simulink model "single_phase_multilevel_sm"  (R2026a)
settings: Solver=ode1be  StopTime=simlength  FixedStep=tc
values from neighbouring files (symbols this model uses):
  Vfc1_base = Udc/5    [plotting_modulation.m]    (also in plotting_results.m; plotting_results_hf.m)
  Vfc2_base = 2*Vfc1_base    [plotting_modulation.m]    (also in plotting_results.m; plotting_results_hf.m)
  Vfc3_base = 3*Vfc1_base    [plotting_modulation.m]    (also in plotting_results.m; plotting_results_hf.m)
  Vfc4_base = 4*Vfc1_base    [plotting_modulation.m]    (also in plotting_results.m; plotting_results_hf.m)
undefined symbols (not defined in the file or in its folder): g0_4Hz, g1_4Hz, I_FS, kalman_omega, kalman_theta, ki_i_inv, ki_v_inv, kp_i_inv, kp_v_inv, Lconn, LFu1, m_dead_time, m_duty_open_loop, magnitude, n1, n10, omega_ref, phase_shift_mod11, phase_shift_mod21, phase_shift_mod31, phase_shift_mod41, phase_shift_mod51, precharge_off, q1kalman, q2kalman, Rbalance, Rconn, RFu, Rkalman, RLFu1, tc, time_pwm_enable, tPWM, ts, V_FS, VCFc_5_init, Vgate_base
libraries: fl_lib x103, nesl_utility x61, simulink x1
(part 1 of 3)
settings Model: SimulationMode=accelerator  Creator=dbagn  LastModifiedBy=dbagn
settings SimscapeCC: SimscapeNominalValues="[{\"value\":\"1\",\"unit\":\"A\"},{\"value\":\"1\",\"unit\":\"bar\"},{\"value\":\"1\",\"unit\":\"cm^2\"},{\"value\":\"1\",\"unit\":\"cm^3/s\"},{\"value\":\"1\",\"unit\":\"kJ/kg\"},{\"value\":\"1\",\"unit\":\"kW\"},{\"value\":\"1\",\"unit\":\"l\"},{\"value\":\"1\",\"unit\":\"N\"},{\"value\":\"1\",\"unit\":\"N*m\"},{\"value\":\"1\",\"unit\":\"V\"}]"  SimscapeLogType=none  SimscapeLogDataHistory=5000.0

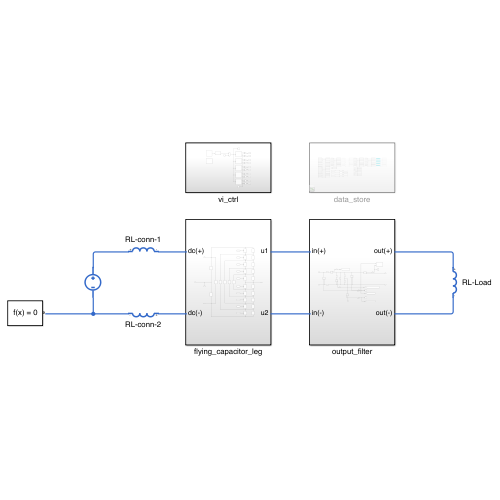
[thumbnail: Simulink's stored preview of the top-level diagram]
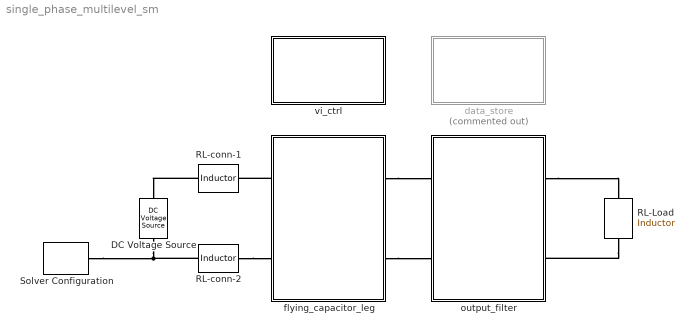
== system single_phase_multilevel_sm ==
  DC Voltage Source : fl_lib/Electrical/Electrical Sources/DC Voltage Source  v0=Udc V
  RL-Load : fl_lib/Electrical/Electrical Elements/Inductor  l=1e-6 H  r=230^2/600 Ohm  g=1e-9 1/Ohm  i_specify=off  i_priority=None  i=0 A  i_nominal_specify=off  i_nominal_value=1  i_nominal_unit=A  v_specify=off  v_priority=None  v=0 V  v_nominal_specify=off  v_nominal_value=1  v_nominal_unit=V  i_L_specify=off  i_L_priority=High  i_L=0 A  i_L_nominal_specify=off  i_L_nominal_value=1  i_L_nominal_unit=A
  RL-conn-1 : fl_lib/Electrical/Electrical Elements/Inductor  l=Lconn/2 H  r=Rconn/2 Ohm  g=1e-9 1/Ohm  i_specify=off  i_priority=None  i=0 A  i_nominal_specify=off  i_nominal_value=1  i_nominal_unit=A  v_specify=off  v_priority=None  v=0 V  v_nominal_specify=off  v_nominal_value=1  v_nominal_unit=V  i_L_specify=off  i_L_priority=High  i_L=0 A  i_L_nominal_specify=off  i_L_nominal_value=1  i_L_nominal_unit=A
  RL-conn-2 : fl_lib/Electrical/Electrical Elements/Inductor  l=Lconn/2 H  r=Rconn/2 Ohm  g=1e-9 1/Ohm  i_specify=off  i_priority=None  i=0 A  i_nominal_specify=off  i_nominal_value=1  i_nominal_unit=A  v_specify=off  v_priority=None  v=0 V  v_nominal_specify=off  v_nominal_value=1  v_nominal_unit=V  i_L_specify=off  i_L_priority=High  i_L=0 A  i_L_nominal_specify=off  i_L_nominal_value=1  i_L_nominal_unit=A
  Solver Configuration : nesl_utility/Solver Configuration  PhysicalDomain=network_engine_domain  SubClassName=solver  LeftPortType=input  RightPortType=generic  Tones=[]  Harmonics=[]  SimulateNoise=off  Profile=off  UseLocalSampling=off  EnableSwitchedLinearOptims=on  FrequencyDomain=off  UseCCode=off  RelTol=0.001  AbsTol=0.001  MinStep=1e-09  ToWorkspace=off  RevertToSquareIcSolve=off  NumHomotopyIterations=100  PhasorMode=off  PhasorModeNumHarmonics=1  ConsistencySolver=NEWTON_XTOL_AFTER_FTOL  CanonicalOrdering=UNORDERED  OptimizeIntermediates=UNOPTIMIZED  IndexReductionMethod=DerivativeReplacement  DoDC=off  ResidualTolerance=1e-09  ConsistencyTolSource=GLOBAL  ConsistencyAbsTol=0.001  ConsistencyRelTol=0.001  ConsistencyTolFactor=0.001  UseLocalSolver=on  LocalSolverChoice=NE_BACKWARD_EULER_ADVANCER  ResolveIndetEquations=on  FunctionEvalNumThread=1  LocalSolverSampleTime=tc  DoFixedCost=on  MaxNonlinIter=3  MaxModeIter=2  ComputeImpulses=off  ImpulseIterations=2  LinearAlgebra=auto  LinearAlgebraNumThread=0  EquationFormulation=NE_TIME_EF  DelaysMemoryBudget=1024  AutomaticFiltering=on  FilteringTimeConstant=0.001  PartitionStorageMethod=AS_NEEDED  PartitionMemoryBudget=1024  PartitionMethod=ROBUST  MultibodyUseLocalSolver=off  MultibodyLocalSolverChoice=ODE1  MultibodyLocalSolverSampleTime=0.001
  data_store : Subsystem  Commented=on
  flying_capacitor_leg : Subsystem
  output_filter : Subsystem
  vi_ctrl : Subsystem
  connections:
  RL-conn-1/LConn1 -- DC Voltage Source/LConn1
  flying_capacitor_leg/RConn1 -- output_filter/LConn1
  output_filter/RConn1 -- RL-Load/LConn1
  RL-Load/RConn1 -- output_filter/RConn2
  flying_capacitor_leg/RConn2 -- output_filter/LConn2
  flying_capacitor_leg/LConn1 -- RL-conn-1/RConn1
  DC Voltage Source/RConn1 -- Solver Configuration/RConn1 -- RL-conn-2/RConn1
  RL-conn-2/LConn1 -- flying_capacitor_leg/LConn2

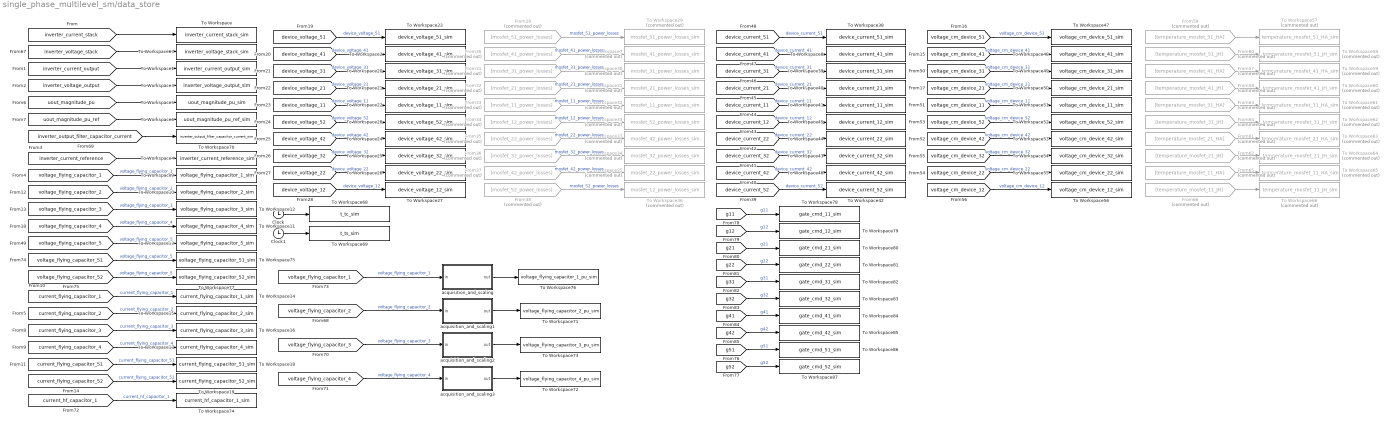
== system single_phase_multilevel_sm/data_store ==
  Clock : Clock
  Clock1 : Clock
  From29 : From  Commented=on  GotoTag=mosfet_51_power_losses  TagVisibility=global
  From30 : From  Commented=on  GotoTag=mosfet_41_power_losses  TagVisibility=global
  From31 : From  Commented=on  GotoTag=mosfet_31_power_losses  TagVisibility=global
  From32 : From  Commented=on  GotoTag=mosfet_21_power_losses  TagVisibility=global
  From33 : From  Commented=on  GotoTag=mosfet_11_power_losses  TagVisibility=global
  From34 : From  Commented=on  GotoTag=mosfet_12_power_losses  TagVisibility=global
  From35 : From  Commented=on  GotoTag=mosfet_22_power_losses  TagVisibility=global
  From36 : From  Commented=on  GotoTag=mosfet_32_power_losses  TagVisibility=global
  From37 : From  Commented=on  GotoTag=mosfet_42_power_losses  TagVisibility=global
  From38 : From  Commented=on  GotoTag=mosfet_52_power_losses  TagVisibility=global
  From57 : From  Commented=on  GotoTag=temperature_mosfet_41_HA  TagVisibility=global
  From58 : From  Commented=on  GotoTag=temperature_mosfet_41_JH  TagVisibility=global
  From59 : From  Commented=on  GotoTag=temperature_mosfet_51_HA  TagVisibility=global
  From60 : From  Commented=on  GotoTag=temperature_mosfet_51_JH  TagVisibility=global
  From61 : From  Commented=on  GotoTag=temperature_mosfet_21_HA  TagVisibility=global
  From62 : From  Commented=on  GotoTag=temperature_mosfet_21_JH  TagVisibility=global
  From63 : From  Commented=on  GotoTag=temperature_mosfet_31_HA  TagVisibility=global
  From64 : From  Commented=on  GotoTag=temperature_mosfet_31_JH  TagVisibility=global
  From65 : From  Commented=on  GotoTag=temperature_mosfet_11_HA  TagVisibility=global
  From66 : From  Commented=on  GotoTag=temperature_mosfet_11_JH  TagVisibility=global
  To Workspace : ToWorkspace  VariableName=inverter_current_stack_sim  SampleTime=tc
      settings: MaxDataPoints=Nc
  To Workspace1 : ToWorkspace  VariableName=inverter_current_output_sim  SampleTime=tc
      settings: MaxDataPoints=Nc
  To Workspace10 : ToWorkspace  VariableName=voltage_flying_capacitor_2_sim  SampleTime=tc
      settings: MaxDataPoints=Nc
  To Workspace11 : ToWorkspace  VariableName=voltage_flying_capacitor_4_sim  SampleTime=tc
      settings: MaxDataPoints=Nc
  To Workspace12 : ToWorkspace  VariableName=voltage_flying_capacitor_3_sim  SampleTime=tc
      settings: MaxDataPoints=Nc
  To Workspace13 : ToWorkspace  VariableName=voltage_flying_capacitor_5_sim  SampleTime=tc
      settings: MaxDataPoints=Nc
  To Workspace14 : ToWorkspace  VariableName=current_flying_capacitor_1_sim  SampleTime=tc
      settings: MaxDataPoints=Nc
  To Workspace15 : ToWorkspace  VariableName=current_flying_capacitor_2_sim  SampleTime=tc
      settings: MaxDataPoints=Nc
  To Workspace16 : ToWorkspace  VariableName=current_flying_capacitor_3_sim  SampleTime=tc
      settings: MaxDataPoints=Nc
  To Workspace17 : ToWorkspace  VariableName=current_flying_capacitor_4_sim  SampleTime=tc
      settings: MaxDataPoints=Nc
  To Workspace18 : ToWorkspace  VariableName=current_flying_capacitor_51_sim  SampleTime=tc
      settings: MaxDataPoints=Nc
  To Workspace19 : ToWorkspace  VariableName=current_flying_capacitor_52_sim  SampleTime=tc
      settings: MaxDataPoints=Nc
  To Workspace2 : ToWorkspace  VariableName=device_voltage_41_sim  SampleTime=tc
      settings: MaxDataPoints=Nc
  To Workspace20 : ToWorkspace  VariableName=device_voltage_31_sim  SampleTime=tc
      settings: MaxDataPoints=Nc
  To Workspace21 : ToWorkspace  VariableName=device_voltage_21_sim  SampleTime=tc
      settings: MaxDataPoints=Nc
  To Workspace22 : ToWorkspace  VariableName=device_voltage_11_sim  SampleTime=tc
      settings: MaxDataPoints=Nc
  To Workspace23 : ToWorkspace  VariableName=device_voltage_51_sim  SampleTime=tc
      settings: MaxDataPoints=Nc
  To Workspace24 : ToWorkspace  VariableName=device_voltage_42_sim  SampleTime=tc
      settings: MaxDataPoints=Nc
  To Workspace25 : ToWorkspace  VariableName=device_voltage_32_sim  SampleTime=tc
      settings: MaxDataPoints=Nc
  To Workspace26 : ToWorkspace  VariableName=device_voltage_22_sim  SampleTime=tc
      settings: MaxDataPoints=Nc
  To Workspace27 : ToWorkspace  VariableName=device_voltage_12_sim  SampleTime=tc
      settings: MaxDataPoints=Nc
  To Workspace28 : ToWorkspace  VariableName=device_voltage_52_sim  SampleTime=tc
      settings: MaxDataPoints=Nc
  To Workspace29 : ToWorkspace  Commented=on  VariableName=mosfet_51_power_losses_sim  SampleTime=tc
      settings: MaxDataPoints=Nc
  To Workspace3 : ToWorkspace  VariableName=inverter_voltage_output_sim  SampleTime=tc
      settings: MaxDataPoints=Nc
  To Workspace30 : ToWorkspace  Commented=on  VariableName=mosfet_31_power_losses_sim  SampleTime=tc
      settings: MaxDataPoints=Nc
  To Workspace31 : ToWorkspace  Commented=on  VariableName=mosfet_21_power_losses_sim  SampleTime=tc
      settings: MaxDataPoints=Nc
  To Workspace32 : ToWorkspace  Commented=on  VariableName=mosfet_11_power_losses_sim  SampleTime=tc
      settings: MaxDataPoints=Nc
  To Workspace33 : ToWorkspace  Commented=on  VariableName=mosfet_52_power_losses_sim  SampleTime=tc
      settings: MaxDataPoints=Nc
  To Workspace34 : ToWorkspace  Commented=on  VariableName=mosfet_32_power_losses_sim  SampleTime=tc
      settings: MaxDataPoints=Nc
  To Workspace35 : ToWorkspace  Commented=on  VariableName=mosfet_22_power_losses_sim  SampleTime=tc
      settings: MaxDataPoints=Nc
  To Workspace36 : ToWorkspace  Commented=on  VariableName=mosfet_12_power_losses_sim  SampleTime=tc
      settings: MaxDataPoints=Nc
  To Workspace37 : ToWorkspace  Commented=on  VariableName=mosfet_42_power_losses_sim  SampleTime=tc
      settings: MaxDataPoints=Nc
  To Workspace38 : ToWorkspace  VariableName=device_current_51_sim  SampleTime=tc
      settings: MaxDataPoints=Nc
  To Workspace39 : ToWorkspace  VariableName=device_current_31_sim  SampleTime=tc
      settings: MaxDataPoints=Nc
  To Workspace4 : ToWorkspace  VariableName=inverter_current_reference_sim  SampleTime=tc
      settings: MaxDataPoints=Nc
  To Workspace40 : ToWorkspace  VariableName=device_current_21_sim  SampleTime=tc
      settings: MaxDataPoints=Nc
  To Workspace41 : ToWorkspace  VariableName=device_current_11_sim  SampleTime=tc
      settings: MaxDataPoints=Nc
  To Workspace42 : ToWorkspace  VariableName=device_current_52_sim  SampleTime=tc
      settings: MaxDataPoints=Nc
  To Workspace43 : ToWorkspace  VariableName=device_current_32_sim  SampleTime=tc
      settings: MaxDataPoints=Nc
  To Workspace44 : ToWorkspace  VariableName=device_current_22_sim  SampleTime=tc
      settings: MaxDataPoints=Nc
  To Workspace45 : ToWorkspace  VariableName=device_current_12_sim  SampleTime=tc
      settings: MaxDataPoints=Nc
  To Workspace46 : ToWorkspace  VariableName=device_current_42_sim  SampleTime=tc
      settings: MaxDataPoints=Nc
  To Workspace47 : ToWorkspace  VariableName=voltage_cm_device_51_sim  SampleTime=tc
      settings: MaxDataPoints=Nc
  To Workspace48 : ToWorkspace  VariableName=voltage_cm_device_41_sim  SampleTime=tc
      settings: MaxDataPoints=Nc
  To Workspace49 : ToWorkspace  VariableName=voltage_cm_device_31_sim  SampleTime=tc
      settings: MaxDataPoints=Nc
  To Workspace5 : ToWorkspace  VariableName=uout_magnitude_pu_sim  SampleTime=tc
      settings: MaxDataPoints=Nc
  To Workspace50 : ToWorkspace  VariableName=voltage_cm_device_21_sim  SampleTime=tc
      settings: MaxDataPoints=Nc
  To Workspace51 : ToWorkspace  VariableName=voltage_cm_device_11_sim  SampleTime=tc
      settings: MaxDataPoints=Nc
  To Workspace52 : ToWorkspace  VariableName=voltage_cm_device_52_sim  SampleTime=tc
      settings: MaxDataPoints=Nc
  To Workspace53 : ToWorkspace  VariableName=voltage_cm_device_42_sim  SampleTime=tc
      settings: MaxDataPoints=Nc
  To Workspace54 : ToWorkspace  VariableName=voltage_cm_device_32_sim  SampleTime=tc
      settings: MaxDataPoints=Nc
  To Workspace55 : ToWorkspace  VariableName=voltage_cm_device_22_sim  SampleTime=tc
      settings: MaxDataPoints=Nc
  To Workspace56 : ToWorkspace  VariableName=voltage_cm_device_12_sim  SampleTime=tc
      settings: MaxDataPoints=Nc
  To Workspace57 : ToWorkspace  Commented=on  VariableName=temperature_mosfet_51_HA_sim  SampleTime=ts
      settings: MaxDataPoints=Ns
  To Workspace58 : ToWorkspace  Commented=on  VariableName=temperature_mosfet_51_JH_sim  SampleTime=ts
      settings: MaxDataPoints=Ns
  To Workspace59 : ToWorkspace  Commented=on  VariableName=temperature_mosfet_41_HA_sim  SampleTime=ts
      settings: MaxDataPoints=Ns
  To Workspace6 : ToWorkspace  VariableName=uout_magnitude_pu_ref_sim  SampleTime=tc
      settings: MaxDataPoints=Nc
  To Workspace60 : ToWorkspace  Commented=on  VariableName=temperature_mosfet_41_JH_sim  SampleTime=ts
      settings: MaxDataPoints=Ns
  To Workspace61 : ToWorkspace  Commented=on  VariableName=temperature_mosfet_31_HA_sim  SampleTime=ts
      settings: MaxDataPoints=Ns
  To Workspace62 : ToWorkspace  Commented=on  VariableName=temperature_mosfet_31_JH_sim  SampleTime=ts
      settings: MaxDataPoints=Ns
  To Workspace63 : ToWorkspace  Commented=on  VariableName=temperature_mosfet_21_HA_sim  SampleTime=ts
      settings: MaxDataPoints=Ns
  To Workspace64 : ToWorkspace  Commented=on  VariableName=temperature_mosfet_21_JH_sim  SampleTime=ts
      settings: MaxDataPoints=Ns
  To Workspace65 : ToWorkspace  Commented=on  VariableName=temperature_mosfet_11_HA_sim  SampleTime=ts
      settings: MaxDataPoints=Ns
  To Workspace66 : ToWorkspace  Commented=on  VariableName=temperature_mosfet_11_JH_sim  SampleTime=ts
      settings: MaxDataPoints=Ns
  To Workspace67 : ToWorkspace  VariableName=inverter_voltage_stack_sim  SampleTime=tc
      settings: MaxDataPoints=Nc
  To Workspace68 : ToWorkspace  VariableName=t_tc_sim  SampleTime=tc
      settings: MaxDataPoints=Nc
  To Workspace69 : ToWorkspace  VariableName=t_ts_sim  SampleTime=ts
      settings: MaxDataPoints=Ns
  To Workspace7 : ToWorkspace  Commented=on  VariableName=mosfet_41_power_losses_sim  SampleTime=tc
      settings: MaxDataPoints=Nc
  To Workspace70 : ToWorkspace  VariableName=inverter_output_filter_capacitor_current_sim  SampleTime=tc
      settings: MaxDataPoints=Nc
  To Workspace71 : ToWorkspace  VariableName=voltage_flying_capacitor_2_pu_sim  SampleTime=ts
      settings: MaxDataPoints=Ns
  To Workspace72 : ToWorkspace  VariableName=voltage_flying_capacitor_4_pu_sim  SampleTime=ts
      settings: MaxDataPoints=Ns
  To Workspace73 : ToWorkspace  VariableName=voltage_flying_capacitor_3_pu_sim  SampleTime=ts
      settings: MaxDataPoints=Ns
  To Workspace74 : ToWorkspace  VariableName=current_hf_capacitor_1_sim  SampleTime=tc
      settings: MaxDataPoints=Nc
  To Workspace75 : ToWorkspace  VariableName=voltage_flying_capacitor_51_sim  SampleTime=tc
      settings: MaxDataPoints=Nc
  To Workspace76 : ToWorkspace  VariableName=voltage_flying_capacitor_1_pu_sim  SampleTime=ts
      settings: MaxDataPoints=Ns
  To Workspace77 : ToWorkspace  VariableName=voltage_flying_capacitor_52_sim  SampleTime=tc
      settings: MaxDataPoints=Nc
  To Workspace78 : ToWorkspace  VariableName=gate_cmd_11_sim  SampleTime=tc
      settings: MaxDataPoints=Nc
  To Workspace79 : ToWorkspace  VariableName=gate_cmd_12_sim  SampleTime=tc
      settings: MaxDataPoints=Nc
  To Workspace8 : ToWorkspace  VariableName=device_current_41_sim  SampleTime=tc
      settings: MaxDataPoints=Nc
  To Workspace80 : ToWorkspace  VariableName=gate_cmd_21_sim  SampleTime=tc
      settings: MaxDataPoints=Nc
  To Workspace81 : ToWorkspace  VariableName=gate_cmd_22_sim  SampleTime=tc
      settings: MaxDataPoints=Nc
  To Workspace82 : ToWorkspace  VariableName=gate_cmd_31_sim  SampleTime=tc
      settings: MaxDataPoints=Nc
  To Workspace83 : ToWorkspace  VariableName=gate_cmd_32_sim  SampleTime=tc
      settings: MaxDataPoints=Nc
  To Workspace84 : ToWorkspace  VariableName=gate_cmd_41_sim  SampleTime=tc
      settings: MaxDataPoints=Nc
  To Workspace85 : ToWorkspace  VariableName=gate_cmd_42_sim  SampleTime=tc
      settings: MaxDataPoints=Nc
  To Workspace86 : ToWorkspace  VariableName=gate_cmd_51_sim  SampleTime=tc
      settings: MaxDataPoints=Nc
  To Workspace87 : ToWorkspace  VariableName=gate_cmd_52_sim  SampleTime=tc
      settings: MaxDataPoints=Nc
  To Workspace9 : ToWorkspace  VariableName=voltage_flying_capacitor_1_sim  SampleTime=tc
      settings: MaxDataPoints=Nc
  acquisition_and_scaling : Subsystem
  acquisition_and_scaling1 : Subsystem
  acquisition_and_scaling2 : Subsystem
  acquisition_and_scaling3 : Subsystem
  wires:
  [inverter_current_stack] -> To Workspace/1
  [inverter_current_output] -> To Workspace1/1
  [inverter_voltage_output] -> To Workspace3/1
  [uout_magnitude_pu] -> To Workspace5/1
  [inverter_current_reference] -> To Workspace4/1
  [uout_magnitude_pu_ref] -> To Workspace6/1
  From30/1 -> To Workspace7/1  "mosfet_41_power_losses"
  [device_voltage_41] -> To Workspace2/1  "device_voltage_41"
  [device_current_41] -> To Workspace8/1  "device_current_41"
  [voltage_flying_capacitor_1] -> To Workspace9/1  "voltage_flying_capacitor_1"
  [voltage_flying_capacitor_2] -> To Workspace10/1  "voltage_flying_capacitor_2"
  [voltage_flying_capacitor_3] -> To Workspace12/1  "voltage_flying_capacitor_3"
  [voltage_flying_capacitor_4] -> To Workspace11/1  "voltage_flying_capacitor_4"
  [voltage_flying_capacitor_5] -> To Workspace13/1  "voltage_flying_capacitor_5"
  [current_flying_capacitor_1] -> To Workspace14/1  "current_flying_capacitor_1"
  [current_flying_capacitor_2] -> To Workspace15/1  "current_flying_capacitor_2"
  [current_flying_capacitor_3] -> To Workspace16/1  "current_flying_capacitor_3"
  [current_flying_capacitor_4] -> To Workspace17/1  "current_flying_capacitor_4"
  [current_flying_capacitor_51] -> To Workspace18/1  "current_flying_capacitor_51"
  [current_flying_capacitor_52] -> To Workspace19/1  "current_flying_capacitor_52"
  [device_voltage_31] -> To Workspace20/1  "device_voltage_31"
  [device_voltage_21] -> To Workspace21/1  "device_voltage_21"
  [device_voltage_11] -> To Workspace22/1  "device_voltage_11"
  [device_voltage_51] -> To Workspace23/1  "device_voltage_51"
  [device_voltage_52] -> To Workspace28/1  "device_voltage_52"
  [device_voltage_42] -> To Workspace24/1  "device_voltage_42"
  [device_voltage_32] -> To Workspace25/1  "device_voltage_32"
  [device_voltage_22] -> To Workspace26/1  "device_voltage_22"
  [device_voltage_12] -> To Workspace27/1  "device_voltage_12"
  From29/1 -> To Workspace29/1  "mosfet_51_power_losses"
  From31/1 -> To Workspace30/1  "mosfet_31_power_losses"
  From32/1 -> To Workspace31/1  "mosfet_21_power_losses"
  From33/1 -> To Workspace32/1  "mosfet_11_power_losses"
  From38/1 -> To Workspace36/1  "mosfet_52_power_losses"
  From37/1 -> To Workspace35/1  "mosfet_42_power_losses"
  From36/1 -> To Workspace34/1  "mosfet_32_power_losses"
  From35/1 -> To Workspace37/1  "mosfet_22_power_losses"
  From34/1 -> To Workspace33/1  "mosfet_12_power_losses"
  [device_current_51] -> To Workspace38/1  "device_current_51"
  [device_current_21] -> To Workspace40/1  "device_current_21"
  [device_current_31] -> To Workspace39/1  "device_current_31"
  [device_current_11] -> To Workspace41/1  "device_current_11"
  [device_current_12] -> To Workspace45/1  "device_current_12"
  [device_current_22] -> To Workspace44/1  "device_current_22"
  [device_current_32] -> To Workspace43/1  "device_current_32"
  [device_current_42] -> To Workspace46/1  "device_current_42"
  [device_current_52] -> To Workspace42/1  "device_current_52"
  [voltage_cm_device_51] -> To Workspace47/1  "voltage_cm_device_51"
  [voltage_cm_device_41] -> To Workspace48/1  "voltage_cm_device_41"
  [voltage_cm_device_21] -> To Workspace50/1  "voltage_cm_device_21"
  [voltage_cm_device_31] -> To Workspace49/1  "voltage_cm_device_31"
  [voltage_cm_device_11] -> To Workspace51/1  "voltage_cm_device_11"
  [voltage_cm_device_12] -> To Workspace56/1  "voltage_cm_device_12"
  [voltage_cm_device_32] -> To Workspace54/1  "voltage_cm_device_32"
  [voltage_cm_device_22] -> To Workspace55/1  "voltage_cm_device_22"
  [voltage_cm_device_42] -> To Workspace53/1  "voltage_cm_device_42"
  [voltage_cm_device_52] -> To Workspace52/1  "voltage_cm_device_52"
  From59/1 -> To Workspace57/1
  From60/1 -> To Workspace58/1
  From58/1 -> To Workspace60/1
  From57/1 -> To Workspace59/1
  From61/1 -> To Workspace63/1
  From62/1 -> To Workspace64/1
  From64/1 -> To Workspace62/1
  From63/1 -> To Workspace61/1
  From66/1 -> To Workspace66/1
  From65/1 -> To Workspace65/1
  [inverter_voltage_stack] -> To Workspace67/1
  Clock/1 -> To Workspace68/1
  Clock1/1 -> To Workspace69/1
  [inverter_output_filter_capacitor_current] -> To Workspace70/1
  [voltage_flying_capacitor_4] -> acquisition_and_scaling3/1(in)  "voltage_flying_capacitor_4"
  [voltage_flying_capacitor_3] -> acquisition_and_scaling2/1(in)  "voltage_flying_capacitor_3"
  [voltage_flying_capacitor_2] -> acquisition_and_scaling1/1(in)  "voltage_flying_capacitor_2"
  [voltage_flying_capacitor_1] -> acquisition_and_scaling/1(in)  "voltage_flying_capacitor_1"
  acquisition_and_scaling/1(out) -> To Workspace76/1
  acquisition_and_scaling1/1(out) -> To Workspace71/1
  acquisition_and_scaling2/1(out) -> To Workspace73/1
  acquisition_and_scaling3/1(out) -> To Workspace72/1
  [current_hf_capacitor_1] -> To Workspace74/1  "current_hf_capacitor_1"
  [voltage_flying_capacitor_51] -> To Workspace75/1  "voltage_flying_capacitor_5"
  [voltage_flying_capacitor_52] -> To Workspace77/1  "voltage_flying_capacitor_5"
  [g11] -> To Workspace78/1  "g11"
  [g12] -> To Workspace79/1  "g12"
  [g21] -> To Workspace80/1  "g21"
  [g22] -> To Workspace81/1  "g22"
  [g31] -> To Workspace82/1  "g31"
  [g32] -> To Workspace83/1  "g32"
  [g41] -> To Workspace84/1  "g41"
  [g42] -> To Workspace85/1  "g42"
  [g51] -> To Workspace86/1  "g51"
  [g52] -> To Workspace87/1  "g52"

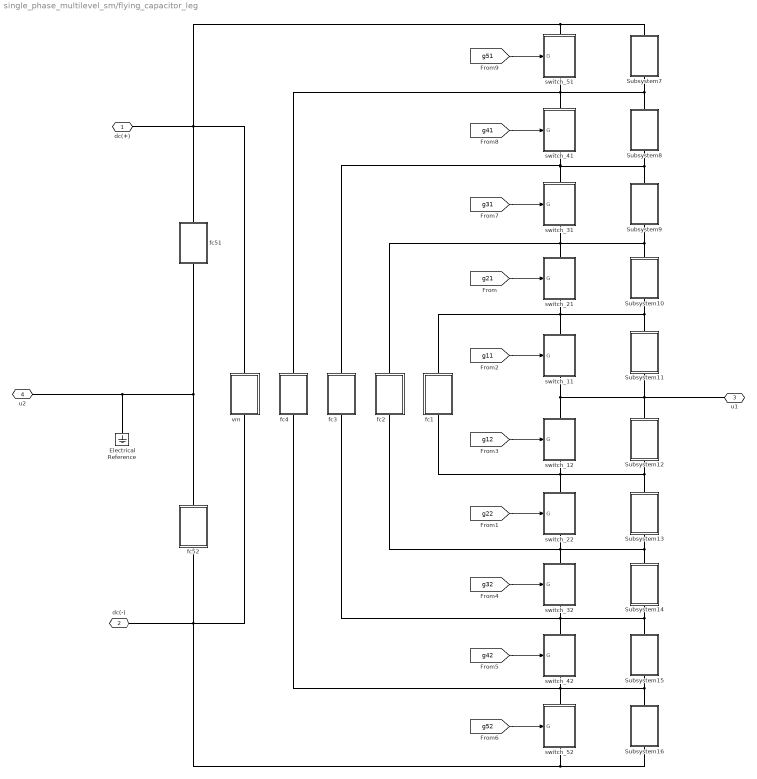
== system single_phase_multilevel_sm/flying_capacitor_leg ==
  Electrical Reference : fl_lib/Electrical/Electrical Elements/Electrical Reference
  Subsystem10 : Subsystem
  Subsystem11 : Subsystem
  Subsystem12 : Subsystem
  Subsystem13 : Subsystem
  Subsystem14 : Subsystem
  Subsystem15 : Subsystem
  Subsystem16 : Subsystem
  Subsystem7 : Subsystem
  Subsystem8 : Subsystem
  Subsystem9 : Subsystem
  fc1 : Subsystem
  fc2 : Subsystem
  fc3 : Subsystem
  fc4 : Subsystem
  fc51 : Subsystem
  fc52 : Subsystem
  switch_11 : Subsystem
      settings: PortSchema="{\"entries\":[{\"content\":{\"sides\":[{\"content\":{\"connectorIds\":[\"In1\"]},\"type\":\"ConnectorPlacement.EquallySpacedRectSide\",\"uuid\":\"e5eb357e-e6a3-4597-845e-75ccc7408620\"},{\"content\":{\"side\":\"RIGHT\"},\"type\":\"ConnectorPlacement.EquallySpacedRectSide\",\"uuid\":\"ee3327c3-644e-4e44-80c9-5d4aeed05850\"},{\"content\":{\"connectorIds\":[\"LConn1\"],\"side\":\"TOP\"},\"type\":\"ConnectorPlacement.EquallySpacedRectSide\",\"uuid\":\"098c4288-4784-4616-bbed-3e6146c90f38\"},{\"content\":{\"connectorIds\":[\"RConn1\"],\"side\":\"BOTTOM\"},\"type\":\"ConnectorPlacement.EquallySpacedRectSide\",\"uuid\":\"c082d048-699c-40cc-b498-4cf10dbd4d73\"}]},\"type\":\"ConnectorPlacement.EquallySpacedConnector\",\"uuid\":\"7fa25437-4a05-4b62-8f9a-bed0c8f2aa7e\"}],\"packageUris\":[\"http://schema.mathworks.com/mf0/Connector/R2020b\"],\"version\":\"1.0\"}"
  switch_12 : Subsystem
      settings: PortSchema="{\"entries\":[{\"content\":{\"sides\":[{\"content\":{\"connectorIds\":[\"In1\"]},\"type\":\"ConnectorPlacement.EquallySpacedRectSide\",\"uuid\":\"e5eb357e-e6a3-4597-845e-75ccc7408620\"},{\"content\":{\"side\":\"RIGHT\"},\"type\":\"ConnectorPlacement.EquallySpacedRectSide\",\"uuid\":\"ee3327c3-644e-4e44-80c9-5d4aeed05850\"},{\"content\":{\"connectorIds\":[\"LConn1\"],\"side\":\"TOP\"},\"type\":\"ConnectorPlacement.EquallySpacedRectSide\",\"uuid\":\"098c4288-4784-4616-bbed-3e6146c90f38\"},{\"content\":{\"connectorIds\":[\"RConn1\"],\"side\":\"BOTTOM\"},\"type\":\"ConnectorPlacement.EquallySpacedRectSide\",\"uuid\":\"c082d048-699c-40cc-b498-4cf10dbd4d73\"}]},\"type\":\"ConnectorPlacement.EquallySpacedConnector\",\"uuid\":\"7fa25437-4a05-4b62-8f9a-bed0c8f2aa7e\"}],\"packageUris\":[\"http://schema.mathworks.com/mf0/Connector/R2020b\"],\"version\":\"1.0\"}"
  switch_21 : Subsystem
      settings: PortSchema="{\"entries\":[{\"content\":{\"sides\":[{\"content\":{\"connectorIds\":[\"In1\"]},\"type\":\"ConnectorPlacement.EquallySpacedRectSide\",\"uuid\":\"e5eb357e-e6a3-4597-845e-75ccc7408620\"},{\"content\":{\"side\":\"RIGHT\"},\"type\":\"ConnectorPlacement.EquallySpacedRectSide\",\"uuid\":\"ee3327c3-644e-4e44-80c9-5d4aeed05850\"},{\"content\":{\"connectorIds\":[\"LConn1\"],\"side\":\"TOP\"},\"type\":\"ConnectorPlacement.EquallySpacedRectSide\",\"uuid\":\"098c4288-4784-4616-bbed-3e6146c90f38\"},{\"content\":{\"connectorIds\":[\"RConn1\"],\"side\":\"BOTTOM\"},\"type\":\"ConnectorPlacement.EquallySpacedRectSide\",\"uuid\":\"c082d048-699c-40cc-b498-4cf10dbd4d73\"}]},\"type\":\"ConnectorPlacement.EquallySpacedConnector\",\"uuid\":\"7fa25437-4a05-4b62-8f9a-bed0c8f2aa7e\"}],\"packageUris\":[\"http://schema.mathworks.com/mf0/Connector/R2020b\"],\"version\":\"1.0\"}"
  switch_22 : Subsystem
      settings: PortSchema="{\"entries\":[{\"content\":{\"sides\":[{\"content\":{\"connectorIds\":[\"In1\"]},\"type\":\"ConnectorPlacement.EquallySpacedRectSide\",\"uuid\":\"e5eb357e-e6a3-4597-845e-75ccc7408620\"},{\"content\":{\"side\":\"RIGHT\"},\"type\":\"ConnectorPlacement.EquallySpacedRectSide\",\"uuid\":\"ee3327c3-644e-4e44-80c9-5d4aeed05850\"},{\"content\":{\"connectorIds\":[\"LConn1\"],\"side\":\"TOP\"},\"type\":\"ConnectorPlacement.EquallySpacedRectSide\",\"uuid\":\"098c4288-4784-4616-bbed-3e6146c90f38\"},{\"content\":{\"connectorIds\":[\"RConn1\"],\"side\":\"BOTTOM\"},\"type\":\"ConnectorPlacement.EquallySpacedRectSide\",\"uuid\":\"c082d048-699c-40cc-b498-4cf10dbd4d73\"}]},\"type\":\"ConnectorPlacement.EquallySpacedConnector\",\"uuid\":\"7fa25437-4a05-4b62-8f9a-bed0c8f2aa7e\"}],\"packageUris\":[\"http://schema.mathworks.com/mf0/Connector/R2020b\"],\"version\":\"1.0\"}"
  switch_31 : Subsystem
      settings: PortSchema="{\"entries\":[{\"content\":{\"sides\":[{\"content\":{\"connectorIds\":[\"In1\"]},\"type\":\"ConnectorPlacement.EquallySpacedRectSide\",\"uuid\":\"e5eb357e-e6a3-4597-845e-75ccc7408620\"},{\"content\":{\"side\":\"RIGHT\"},\"type\":\"ConnectorPlacement.EquallySpacedRectSide\",\"uuid\":\"ee3327c3-644e-4e44-80c9-5d4aeed05850\"},{\"content\":{\"connectorIds\":[\"LConn1\"],\"side\":\"TOP\"},\"type\":\"ConnectorPlacement.EquallySpacedRectSide\",\"uuid\":\"098c4288-4784-4616-bbed-3e6146c90f38\"},{\"content\":{\"connectorIds\":[\"RConn1\"],\"side\":\"BOTTOM\"},\"type\":\"ConnectorPlacement.EquallySpacedRectSide\",\"uuid\":\"c082d048-699c-40cc-b498-4cf10dbd4d73\"}]},\"type\":\"ConnectorPlacement.EquallySpacedConnector\",\"uuid\":\"7fa25437-4a05-4b62-8f9a-bed0c8f2aa7e\"}],\"packageUris\":[\"http://schema.mathworks.com/mf0/Connector/R2020b\"],\"version\":\"1.0\"}"
  switch_32 : Subsystem
      settings: PortSchema="{\"entries\":[{\"content\":{\"sides\":[{\"content\":{\"connectorIds\":[\"In1\"]},\"type\":\"ConnectorPlacement.EquallySpacedRectSide\",\"uuid\":\"e5eb357e-e6a3-4597-845e-75ccc7408620\"},{\"content\":{\"side\":\"RIGHT\"},\"type\":\"ConnectorPlacement.EquallySpacedRectSide\",\"uuid\":\"ee3327c3-644e-4e44-80c9-5d4aeed05850\"},{\"content\":{\"connectorIds\":[\"LConn1\"],\"side\":\"TOP\"},\"type\":\"ConnectorPlacement.EquallySpacedRectSide\",\"uuid\":\"098c4288-4784-4616-bbed-3e6146c90f38\"},{\"content\":{\"connectorIds\":[\"RConn1\"],\"side\":\"BOTTOM\"},\"type\":\"ConnectorPlacement.EquallySpacedRectSide\",\"uuid\":\"c082d048-699c-40cc-b498-4cf10dbd4d73\"}]},\"type\":\"ConnectorPlacement.EquallySpacedConnector\",\"uuid\":\"7fa25437-4a05-4b62-8f9a-bed0c8f2aa7e\"}],\"packageUris\":[\"http://schema.mathworks.com/mf0/Connector/R2020b\"],\"version\":\"1.0\"}"
  switch_41 : Subsystem
      settings: PortSchema="{\"entries\":[{\"content\":{\"sides\":[{\"content\":{\"connectorIds\":[\"In1\"]},\"type\":\"ConnectorPlacement.EquallySpacedRectSide\",\"uuid\":\"e5eb357e-e6a3-4597-845e-75ccc7408620\"},{\"content\":{\"side\":\"RIGHT\"},\"type\":\"ConnectorPlacement.EquallySpacedRectSide\",\"uuid\":\"ee3327c3-644e-4e44-80c9-5d4aeed05850\"},{\"content\":{\"connectorIds\":[\"LConn1\"],\"side\":\"TOP\"},\"type\":\"ConnectorPlacement.EquallySpacedRectSide\",\"uuid\":\"098c4288-4784-4616-bbed-3e6146c90f38\"},{\"content\":{\"connectorIds\":[\"RConn1\"],\"side\":\"BOTTOM\"},\"type\":\"ConnectorPlacement.EquallySpacedRectSide\",\"uuid\":\"c082d048-699c-40cc-b498-4cf10dbd4d73\"}]},\"type\":\"ConnectorPlacement.EquallySpacedConnector\",\"uuid\":\"7fa25437-4a05-4b62-8f9a-bed0c8f2aa7e\"}],\"packageUris\":[\"http://schema.mathworks.com/mf0/Connector/R2020b\"],\"version\":\"1.0\"}"
  switch_42 : Subsystem
      settings: PortSchema="{\"entries\":[{\"content\":{\"sides\":[{\"content\":{\"connectorIds\":[\"In1\"]},\"type\":\"ConnectorPlacement.EquallySpacedRectSide\",\"uuid\":\"e5eb357e-e6a3-4597-845e-75ccc7408620\"},{\"content\":{\"side\":\"RIGHT\"},\"type\":\"ConnectorPlacement.EquallySpacedRectSide\",\"uuid\":\"ee3327c3-644e-4e44-80c9-5d4aeed05850\"},{\"content\":{\"connectorIds\":[\"LConn1\"],\"side\":\"TOP\"},\"type\":\"ConnectorPlacement.EquallySpacedRectSide\",\"uuid\":\"098c4288-4784-4616-bbed-3e6146c90f38\"},{\"content\":{\"connectorIds\":[\"RConn1\"],\"side\":\"BOTTOM\"},\"type\":\"ConnectorPlacement.EquallySpacedRectSide\",\"uuid\":\"c082d048-699c-40cc-b498-4cf10dbd4d73\"}]},\"type\":\"ConnectorPlacement.EquallySpacedConnector\",\"uuid\":\"7fa25437-4a05-4b62-8f9a-bed0c8f2aa7e\"}],\"packageUris\":[\"http://schema.mathworks.com/mf0/Connector/R2020b\"],\"version\":\"1.0\"}"
  switch_51 : Subsystem
      settings: PortSchema="{\"entries\":[{\"content\":{\"sides\":[{\"content\":{\"connectorIds\":[\"In1\"]},\"type\":\"ConnectorPlacement.EquallySpacedRectSide\",\"uuid\":\"e5eb357e-e6a3-4597-845e-75ccc7408620\"},{\"content\":{\"side\":\"RIGHT\"},\"type\":\"ConnectorPlacement.EquallySpacedRectSide\",\"uuid\":\"ee3327c3-644e-4e44-80c9-5d4aeed05850\"},{\"content\":{\"connectorIds\":[\"LConn1\"],\"side\":\"TOP\"},\"type\":\"ConnectorPlacement.EquallySpacedRectSide\",\"uuid\":\"098c4288-4784-4616-bbed-3e6146c90f38\"},{\"content\":{\"connectorIds\":[\"RConn1\"],\"side\":\"BOTTOM\"},\"type\":\"ConnectorPlacement.EquallySpacedRectSide\",\"uuid\":\"c082d048-699c-40cc-b498-4cf10dbd4d73\"}]},\"type\":\"ConnectorPlacement.EquallySpacedConnector\",\"uuid\":\"7fa25437-4a05-4b62-8f9a-bed0c8f2aa7e\"}],\"packageUris\":[\"http://schema.mathworks.com/mf0/Connector/R2020b\"],\"version\":\"1.0\"}"
  switch_52 : Subsystem
      settings: PortSchema="{\"entries\":[{\"content\":{\"sides\":[{\"content\":{\"connectorIds\":[\"In1\"]},\"type\":\"ConnectorPlacement.EquallySpacedRectSide\",\"uuid\":\"e5eb357e-e6a3-4597-845e-75ccc7408620\"},{\"content\":{\"side\":\"RIGHT\"},\"type\":\"ConnectorPlacement.EquallySpacedRectSide\",\"uuid\":\"ee3327c3-644e-4e44-80c9-5d4aeed05850\"},{\"content\":{\"connectorIds\":[\"LConn1\"],\"side\":\"TOP\"},\"type\":\"ConnectorPlacement.EquallySpacedRectSide\",\"uuid\":\"098c4288-4784-4616-bbed-3e6146c90f38\"},{\"content\":{\"connectorIds\":[\"RConn1\"],\"side\":\"BOTTOM\"},\"type\":\"ConnectorPlacement.EquallySpacedRectSide\",\"uuid\":\"c082d048-699c-40cc-b498-4cf10dbd4d73\"}]},\"type\":\"ConnectorPlacement.EquallySpacedConnector\",\"uuid\":\"7fa25437-4a05-4b62-8f9a-bed0c8f2aa7e\"}],\"packageUris\":[\"http://schema.mathworks.com/mf0/Connector/R2020b\"],\"version\":\"1.0\"}"
  vm : Subsystem
  dc(+) : PMIOPort  Side=Left
  dc(-) : PMIOPort  Port=2  Side=Left
  u1 : PMIOPort  Port=3  Side=Right
  u2 : PMIOPort  Port=4  Side=Right
  wires:
  [g22] -> switch_22/1(G)
  [g21] -> switch_21/1(G)
  [g11] -> switch_11/1(G)
  [g12] -> switch_12/1(G)
  [g32] -> switch_32/1(G)
  [g42] -> switch_42/1(G)
  [g52] -> switch_52/1(G)
  [g31] -> switch_31/1(G)
  [g41] -> switch_41/1(G)
  [g51] -> switch_51/1(G)
  connections:
  Subsystem7/LConn1 -- fc51/LConn1 -- vm/LConn1 -- dc(+)/RConn1 -- switch_51/LConn1
  switch_52/RConn1 -- Subsystem16/RConn1 -- fc52/RConn1 -- vm/RConn1 -- dc(-)/RConn1
  switch_12/LConn1 -- Subsystem11/RConn1 -- u1/RConn1 -- Subsystem12/LConn1 -- switch_11/RConn1
  fc3/LConn1 -- switch_41/RConn1 -- Subsystem9/LConn1 -- Subsystem8/RConn1 -- switch_31/LConn1
  fc4/LConn1 -- switch_41/LConn1 -- switch_51/RConn1 -- Subsystem8/LConn1 -- Subsystem7/RConn1
  fc2/RConn1 -- Subsystem13/RConn1 -- Subsystem14/LConn1 -- switch_32/LConn1 -- switch_22/RConn1
  switch_12/RConn1 -- Subsystem12/RConn1 -- Subsystem13/LConn1 -- switch_22/LConn1 -- fc1/RConn1
  u2/RConn1 -- Electrical Reference/LConn1 -- fc51/RConn1 -- fc52/LConn1
  switch_52/LConn1 -- Subsystem15/RConn1 -- Subsystem16/LConn1 -- switch_42/RConn1 -- fc4/RConn1
  switch_32/RConn1 -- Subsystem15/LConn1 -- Subsystem14/RConn1 -- switch_42/LConn1 -- fc3/RConn1
  fc2/LConn1 -- Subsystem10/LConn1 -- Subsystem9/RConn1 -- switch_21/LConn1 -- switch_31/RConn1
  switch_11/LConn1 -- Subsystem11/LConn1 -- Subsystem10/RConn1 -- switch_21/RConn1 -- fc1/LConn1

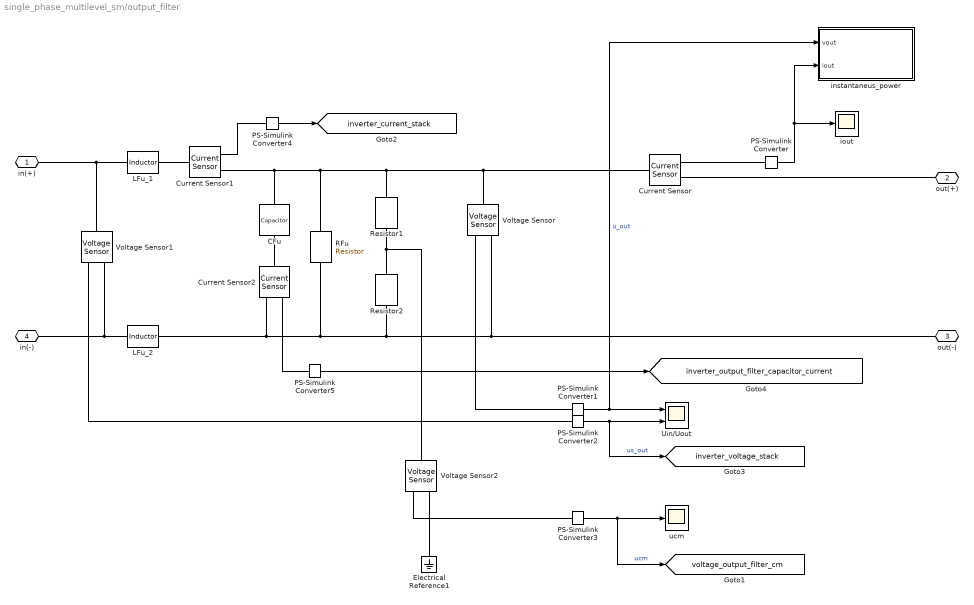
== system single_phase_multilevel_sm/output_filter ==
  CFu : fl_lib/Electrical/Electrical Elements/Capacitor  c=CFu F  r=RCFu Ohm  g=0 1/Ohm  i_specify=off  i_priority=None  i=0 A  i_nominal_specify=off  i_nominal_value=1  i_nominal_unit=A  v_specify=off  v_priority=None  v=0 V  v_nominal_specify=off  v_nominal_value=1  v_nominal_unit=V  vc_specify=off  vc_priority=High  vc=0 V  vc_nominal_specify=off  vc_nominal_value=1  vc_nominal_unit=V
  Current Sensor : fl_lib/Electrical/Electrical Sensors/Current Sensor
  Current Sensor1 : fl_lib/Electrical/Electrical Sensors/Current Sensor
  Current Sensor2 : fl_lib/Electrical/Electrical Sensors/Current Sensor
  Electrical Reference1 : fl_lib/Electrical/Electrical Elements/Electrical Reference
  LFu_1 : fl_lib/Electrical/Electrical Elements/Inductor  l=LFu1/2 H  r=RLFu1/2 Ohm  g=1e-9 1/Ohm  i_specify=off  i_priority=None  i=0 A  i_nominal_specify=off  i_nominal_value=1  i_nominal_unit=A  v_specify=off  v_priority=None  v=0 V  v_nominal_specify=off  v_nominal_value=1  v_nominal_unit=V  i_L_specify=off  i_L_priority=High  i_L=0 A  i_L_nominal_specify=off  i_L_nominal_value=1  i_L_nominal_unit=A
  LFu_2 : fl_lib/Electrical/Electrical Elements/Inductor  l=LFu1/2 H  r=RLFu1/2 Ohm  g=1e-9 1/Ohm  i_specify=off  i_priority=None  i=0 A  i_nominal_specify=off  i_nominal_value=1  i_nominal_unit=A  v_specify=off  v_priority=None  v=0 V  v_nominal_specify=off  v_nominal_value=1  v_nominal_unit=V  i_L_specify=off  i_L_priority=High  i_L=0 A  i_L_nominal_specify=off  i_L_nominal_value=1  i_L_nominal_unit=A
  PS-Simulink Converter : nesl_utility/PS-Simulink Converter  PhysicalDomain=network_engine_domain  SubClassName=ps_output  LeftPortType=input  RightPortType=output  PseudoPeriodic=off  Frequencies=[]  VectorFormat=1-D array  Unit=A  AffineConversion=off
  PS-Simulink Converter1 : nesl_utility/PS-Simulink Converter  PhysicalDomain=network_engine_domain  SubClassName=ps_output  LeftPortType=input  RightPortType=output  PseudoPeriodic=off  Frequencies=[]  VectorFormat=1-D array  Unit=V  AffineConversion=off
  PS-Simulink Converter2 : nesl_utility/PS-Simulink Converter  PhysicalDomain=network_engine_domain  SubClassName=ps_output  LeftPortType=input  RightPortType=output  PseudoPeriodic=off  Frequencies=[]  VectorFormat=1-D array  Unit=V  AffineConversion=off
  PS-Simulink Converter3 : nesl_utility/PS-Simulink Converter  PhysicalDomain=network_engine_domain  SubClassName=ps_output  LeftPortType=input  RightPortType=output  PseudoPeriodic=off  Frequencies=[]  VectorFormat=1-D array  Unit=V  AffineConversion=off
  PS-Simulink Converter4 : nesl_utility/PS-Simulink Converter  PhysicalDomain=network_engine_domain  SubClassName=ps_output  LeftPortType=input  RightPortType=output  PseudoPeriodic=off  Frequencies=[]  VectorFormat=1-D array  Unit=A  AffineConversion=off
  PS-Simulink Converter5 : nesl_utility/PS-Simulink Converter  PhysicalDomain=network_engine_domain  SubClassName=ps_output  LeftPortType=input  RightPortType=output  PseudoPeriodic=off  Frequencies=[]  VectorFormat=1-D array  Unit=A  AffineConversion=off
  RFu : fl_lib/Electrical/Electrical Elements/Resistor  R=RFu Ohm  i_specify=off  i_priority=None  i=0 A  i_nominal_specify=off  i_nominal_value=1  i_nominal_unit=A  v_specify=off  v_priority=None  v=0 V  v_nominal_specify=off  v_nominal_value=1  v_nominal_unit=V
  Resistor1 : fl_lib/Electrical/Electrical Elements/Resistor  R=1e5 Ohm  i_specify=off  i_priority=None  i=0 A  i_nominal_specify=off  i_nominal_value=1  i_nominal_unit=A  v_specify=off  v_priority=None  v=0 V  v_nominal_specify=off  v_nominal_value=1  v_nominal_unit=V
  Resistor2 : fl_lib/Electrical/Electrical Elements/Resistor  R=1e5 Ohm  i_specify=off  i_priority=None  i=0 A  i_nominal_specify=off  i_nominal_value=1  i_nominal_unit=A  v_specify=off  v_priority=None  v=0 V  v_nominal_specify=off  v_nominal_value=1  v_nominal_unit=V
  Uin/Uout : Scope  NumInputPorts=2
      settings: SampleTime=tc  ActiveDisplayYMinimum=-1245.54386  ActiveDisplayYMaximum=1234.03728  DataLoggingVariableName=ScopeData2
  Voltage Sensor : fl_lib/Electrical/Electrical Sensors/Voltage Sensor
  Voltage Sensor1 : fl_lib/Electrical/Electrical Sensors/Voltage Sensor
  Voltage Sensor2 : fl_lib/Electrical/Electrical Sensors/Voltage Sensor
  instantaneus_power : Subsystem
  iout : Scope
      settings: SampleTime=tc  ActiveDisplayYMinimum=-5.781446495004932  ActiveDisplayYMaximum=5.8368797471135245
  ucm : Scope
      settings: SampleTime=tc  ActiveDisplayYMinimum=-621.16944  ActiveDisplayYMaximum=559.37932
  in(+) : PMIOPort  Side=Left
  out(+) : PMIOPort  Port=2  Side=Right
  out(-) : PMIOPort  Port=3  Side=Right
  in(-) : PMIOPort  Port=4  Side=Left
  tag scope: inverter_current_stack=global, inverter_output_filter_capacitor_current=global, inverter_voltage_stack=global, voltage_output_filter_cm=global
  wires:
  PS-Simulink Converter2/1 -> [inverter_voltage_stack], Uin/Uout/2  "us_out"
  PS-Simulink Converter/1 -> iout/1, instantaneus_power/2(iout)
  PS-Simulink Converter3/1 -> [voltage_output_filter_cm], ucm/1  "ucm"
  PS-Simulink Converter4/1 -> [inverter_current_stack]
  PS-Simulink Converter1/1 -> Uin/Uout/1, instantaneus_power/1(vout)  "u_out"
  PS-Simulink Converter5/1 -> [inverter_output_filter_capacitor_current]
  connections:
  out(-)/RConn1 -- Voltage Sensor/RConn2 -- Resistor2/RConn1 -- RFu/RConn1 -- Current Sensor2/RConn2 -- LFu_2/LConn1
  LFu_1/RConn1 -- Current Sensor1/LConn1
  Voltage Sensor1/LConn1 -- LFu_1/LConn1 -- in(+)/RConn1
  PS-Simulink Converter4/LConn1 -- Current Sensor1/RConn1
  Current Sensor/RConn2 -- out(+)/RConn1
  Voltage Sensor2/RConn1 -- PS-Simulink Converter3/LConn1
  Voltage Sensor1/RConn1 -- PS-Simulink Converter2/LConn1
  LFu_2/RConn1 -- in(-)/RConn1 -- Voltage Sensor1/RConn2
  Electrical Reference1/LConn1 -- Voltage Sensor2/RConn2
  Voltage Sensor/RConn1 -- PS-Simulink Converter1/LConn1
  Current Sensor/RConn1 -- PS-Simulink Converter/LConn1
  Current Sensor2/LConn1 -- CFu/RConn1
  Current Sensor2/RConn1 -- PS-Simulink Converter5/LConn1
  CFu/LConn1 -- Current Sensor1/RConn2 -- Resistor1/LConn1 -- Current Sensor/LConn1 -- Voltage Sensor/LConn1 -- RFu/LConn1
  Resistor2/LConn1 -- Voltage Sensor2/LConn1 -- Resistor1/RConn1

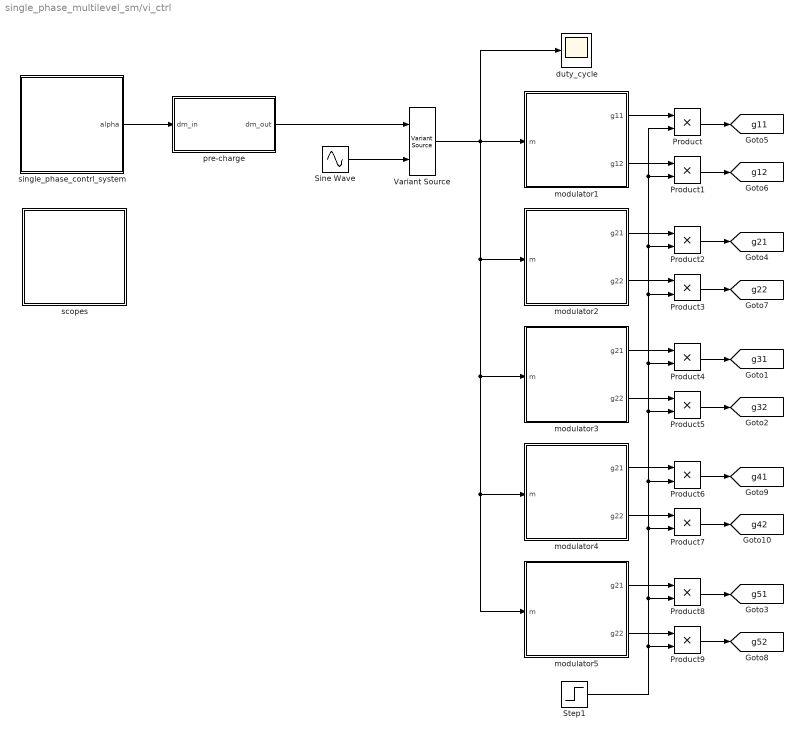
== system single_phase_multilevel_sm/vi_ctrl ==
  Product{,1..9} (10 alike) : Product
  Sine Wave : Sin  Amplitude=m_duty_open_loop  Frequency=2*pi*50  SampleTime=0
  Step1 : Step  Time=time_pwm_enable  SampleTime=0
  Variant Source : VariantSource  VariantControls={enable_high_frequency_analysis == 0, enable_high_frequency_analysis == 1}
  duty_cycle : Scope
      settings: ActiveDisplayYMinimum=-1.25  ActiveDisplayYMaximum=1.25
  modulator1 : Subsystem
  modulator2 : Subsystem
  modulator3 : Subsystem
  modulator4 : Subsystem
  modulator5 : Subsystem
  pre-charge : Subsystem
  scopes : Subsystem
  single_phase_contrl_system : Subsystem
  tag scope: g11=global, g12=global, g21=global, g22=global, g31=global, g32=global, g41=global, g42=global, g51=global, g52=global
  wires:
  modulator1/1(g11) -> Product/1
  modulator1/2(g12) -> Product1/1
  modulator2/1(g21) -> Product2/1
  modulator2/2(g22) -> Product3/1
  modulator3/2(g22) -> Product5/1
  modulator3/1(g21) -> Product4/1
  modulator4/1(g21) -> Product6/1
  modulator4/2(g22) -> Product7/1
  modulator5/1(g21) -> Product8/1
  modulator5/2(g22) -> Product9/1
  Product6/1 -> [g41]
  Product7/1 -> [g42]
  Product8/1 -> [g51]
  Product9/1 -> [g52]
  Product5/1 -> [g32]
  Product4/1 -> [g31]
  Product3/1 -> [g22]
  Product2/1 -> [g21]
  Product1/1 -> [g12]
  Product/1 -> [g11]
  Step1/1 -> Product8/2, Product7/2, Product3/2, Product2/2, Product1/2, Product/2, Product4/2, Product5/2, Product6/2, Product9/2
  Variant Source/1 -> modulator4/1(m), modulator5/1(m), modulator3/1(m), modulator2/1(m), duty_cycle/1, modulator1/1(m)
  single_phase_contrl_system/1(alpha) -> pre-charge/1(dm_in)
  Sine Wave/1 -> Variant Source/2
  pre-charge/1(dm_out) -> Variant Source/1

== system single_phase_multilevel_sm/data_store/acquisition_and_scaling ==
  in : Inport
  1/Ti5 : Gain  Gain=1/Vfc1_base  SaturateOnIntegerOverflow=on  OutDataTypeStr=Inherit: Same as input  ParamDataTypeStr=Inherit: Same as input
  Unit Delay4 : UnitDelay  SampleTime=ts
  Zero-Order Hold1 : ZeroOrderHold  SampleTime=ts
  out : Outport
  wires:
  in/1 -> Zero-Order Hold1/1
  1/Ti5/1 -> Unit Delay4/1
  Zero-Order Hold1/1 -> 1/Ti5/1
  Unit Delay4/1 -> out/1

== system single_phase_multilevel_sm/data_store/acquisition_and_scaling1 ==
  in : Inport
  1/Ti5 : Gain  Gain=1/Vfc2_base  SaturateOnIntegerOverflow=on  OutDataTypeStr=Inherit: Same as input  ParamDataTypeStr=Inherit: Same as input
  Unit Delay4 : UnitDelay  SampleTime=ts
  Zero-Order Hold1 : ZeroOrderHold  SampleTime=ts
  out : Outport
  wires:
  Unit Delay4/1 -> out/1
  Zero-Order Hold1/1 -> 1/Ti5/1
  1/Ti5/1 -> Unit Delay4/1
  in/1 -> Zero-Order Hold1/1

== system single_phase_multilevel_sm/data_store/acquisition_and_scaling2 ==
  in : Inport
  1/Ti5 : Gain  Gain=1/Vfc3_base  SaturateOnIntegerOverflow=on  OutDataTypeStr=Inherit: Same as input  ParamDataTypeStr=Inherit: Same as input
  Unit Delay4 : UnitDelay  SampleTime=ts
  Zero-Order Hold1 : ZeroOrderHold  SampleTime=ts
  out : Outport
  wires:
  in/1 -> Zero-Order Hold1/1
  1/Ti5/1 -> Unit Delay4/1
  Zero-Order Hold1/1 -> 1/Ti5/1
  Unit Delay4/1 -> out/1

== system single_phase_multilevel_sm/data_store/acquisition_and_scaling3 ==
  in : Inport
  1/Ti5 : Gain  Gain=1/Vfc4_base  SaturateOnIntegerOverflow=on  OutDataTypeStr=Inherit: Same as input  ParamDataTypeStr=Inherit: Same as input
  Unit Delay4 : UnitDelay  SampleTime=ts
  Zero-Order Hold1 : ZeroOrderHold  SampleTime=ts
  out : Outport
  wires:
  Unit Delay4/1 -> out/1
  Zero-Order Hold1/1 -> 1/Ti5/1
  1/Ti5/1 -> Unit Delay4/1
  in/1 -> Zero-Order Hold1/1

== system single_phase_multilevel_sm/flying_capacitor_leg/Subsystem10 ==
  Resistor3 : fl_lib/Electrical/Electrical Elements/Resistor  R=Rbalance Ohm  i_specify=off  i_priority=None  i=0 A  i_nominal_specify=off  i_nominal_value=1  i_nominal_unit=A  v_specify=off  v_priority=None  v=0 V  v_nominal_specify=off  v_nominal_value=1  v_nominal_unit=V
  1 : PMIOPort  Side=Left
  2 : PMIOPort  Port=2  Side=Right
  connections:
  Resistor3/LConn1 -- 1/RConn1
  Resistor3/RConn1 -- 2/RConn1

== system single_phase_multilevel_sm/flying_capacitor_leg/Subsystem11 ==
  Resistor3 : fl_lib/Electrical/Electrical Elements/Resistor  R=Rbalance Ohm  i_specify=off  i_priority=None  i=0 A  i_nominal_specify=off  i_nominal_value=1  i_nominal_unit=A  v_specify=off  v_priority=None  v=0 V  v_nominal_specify=off  v_nominal_value=1  v_nominal_unit=V
  1 : PMIOPort  Side=Left
  2 : PMIOPort  Port=2  Side=Right
  connections:
  Resistor3/RConn1 -- 2/RConn1
  Resistor3/LConn1 -- 1/RConn1

== system single_phase_multilevel_sm/flying_capacitor_leg/Subsystem12 ==
  Resistor3 : fl_lib/Electrical/Electrical Elements/Resistor  R=Rbalance Ohm  i_specify=off  i_priority=None  i=0 A  i_nominal_specify=off  i_nominal_value=1  i_nominal_unit=A  v_specify=off  v_priority=None  v=0 V  v_nominal_specify=off  v_nominal_value=1  v_nominal_unit=V
  1 : PMIOPort  Side=Left
  2 : PMIOPort  Port=2  Side=Right
  connections:
  Resistor3/LConn1 -- 1/RConn1
  Resistor3/RConn1 -- 2/RConn1

== system single_phase_multilevel_sm/flying_capacitor_leg/Subsystem13 ==
  Resistor3 : fl_lib/Electrical/Electrical Elements/Resistor  R=Rbalance Ohm  i_specify=off  i_priority=None  i=0 A  i_nominal_specify=off  i_nominal_value=1  i_nominal_unit=A  v_specify=off  v_priority=None  v=0 V  v_nominal_specify=off  v_nominal_value=1  v_nominal_unit=V
  1 : PMIOPort  Side=Left
  2 : PMIOPort  Port=2  Side=Right
  connections:
  Resistor3/RConn1 -- 2/RConn1
  Resistor3/LConn1 -- 1/RConn1

== system single_phase_multilevel_sm/flying_capacitor_leg/Subsystem14 ==
  Resistor3 : fl_lib/Electrical/Electrical Elements/Resistor  R=Rbalance Ohm  i_specify=off  i_priority=None  i=0 A  i_nominal_specify=off  i_nominal_value=1  i_nominal_unit=A  v_specify=off  v_priority=None  v=0 V  v_nominal_specify=off  v_nominal_value=1  v_nominal_unit=V
  1 : PMIOPort  Side=Left
  2 : PMIOPort  Port=2  Side=Right
  connections:
  Resistor3/LConn1 -- 1/RConn1
  Resistor3/RConn1 -- 2/RConn1

== system single_phase_multilevel_sm/flying_capacitor_leg/Subsystem15 ==
  Resistor3 : fl_lib/Electrical/Electrical Elements/Resistor  R=Rbalance Ohm  i_specify=off  i_priority=None  i=0 A  i_nominal_specify=off  i_nominal_value=1  i_nominal_unit=A  v_specify=off  v_priority=None  v=0 V  v_nominal_specify=off  v_nominal_value=1  v_nominal_unit=V
  1 : PMIOPort  Side=Left
  2 : PMIOPort  Port=2  Side=Right
  connections:
  Resistor3/RConn1 -- 2/RConn1
  Resistor3/LConn1 -- 1/RConn1

== system single_phase_multilevel_sm/flying_capacitor_leg/Subsystem16 ==
  Resistor3 : fl_lib/Electrical/Electrical Elements/Resistor  R=Rbalance Ohm  i_specify=off  i_priority=None  i=0 A  i_nominal_specify=off  i_nominal_value=1  i_nominal_unit=A  v_specify=off  v_priority=None  v=0 V  v_nominal_specify=off  v_nominal_value=1  v_nominal_unit=V
  1 : PMIOPort  Side=Left
  2 : PMIOPort  Port=2  Side=Right
  connections:
  Resistor3/LConn1 -- 1/RConn1
  Resistor3/RConn1 -- 2/RConn1

== system single_phase_multilevel_sm/flying_capacitor_leg/Subsystem7 ==
  Resistor3 : fl_lib/Electrical/Electrical Elements/Resistor  R=Rbalance Ohm  i_specify=off  i_priority=None  i=0 A  i_nominal_specify=off  i_nominal_value=1  i_nominal_unit=A  v_specify=off  v_priority=None  v=0 V  v_nominal_specify=off  v_nominal_value=1  v_nominal_unit=V
  1 : PMIOPort  Side=Left
  2 : PMIOPort  Port=2  Side=Right
  connections:
  Resistor3/RConn1 -- 2/RConn1
  Resistor3/LConn1 -- 1/RConn1

== system single_phase_multilevel_sm/flying_capacitor_leg/Subsystem8 ==
  Resistor3 : fl_lib/Electrical/Electrical Elements/Resistor  R=Rbalance Ohm  i_specify=off  i_priority=None  i=0 A  i_nominal_specify=off  i_nominal_value=1  i_nominal_unit=A  v_specify=off  v_priority=None  v=0 V  v_nominal_specify=off  v_nominal_value=1  v_nominal_unit=V
  1 : PMIOPort  Side=Left
  2 : PMIOPort  Port=2  Side=Right
  connections:
  Resistor3/LConn1 -- 1/RConn1
  Resistor3/RConn1 -- 2/RConn1

== system single_phase_multilevel_sm/flying_capacitor_leg/Subsystem9 ==
  Resistor3 : fl_lib/Electrical/Electrical Elements/Resistor  R=Rbalance Ohm  i_specify=off  i_priority=None  i=0 A  i_nominal_specify=off  i_nominal_value=1  i_nominal_unit=A  v_specify=off  v_priority=None  v=0 V  v_nominal_specify=off  v_nominal_value=1  v_nominal_unit=V
  1 : PMIOPort  Side=Left
  2 : PMIOPort  Port=2  Side=Right
  connections:
  Resistor3/RConn1 -- 2/RConn1
  Resistor3/LConn1 -- 1/RConn1
